simulink model "EMRAXDrive"  (R2023a)
settings: Solver=FixedStepAuto  StartTime=0.0  StopTime=emrax.stop_time  FixedStep=(1/6)*10^-05  RelTol=1e-3
PostLoadFcn:
  | motorFolder = fileparts(get_param('EMRAXDrive','FileName'));
  | run(fullfile(motorFolder,'MotorParameters.m'));
  | run(fullfile(motorFolder,'FlightParameters.m'));
  | emrax.flight_step = drone.step_s;
  | emrax.J = emrax.rotor_inertia + emrax.propeller_inertia;
  | emrax.current_limit = sqrt(2)*emrax.continuous_phase_arms; % amplitude-invariant dq, peak A
  | kt = 1.5*emrax.pole_pairs*emrax.flux;
  | current_bw = 2*pi*emrax.fsw/10;
  | inverter_gain = emrax.Vdc/2;
  | emrax.kp_d = current_bw*emrax.Ld/inverter_gain;
  | emrax.kp_q = current_bw*emrax.Lq/inverter_gain;
  | emrax.ki_i = current_bw*emrax.Rs/inverter_gain;
  | a = tand(65) + 1/cosd(65);
  | emrax.tau_filter = 1/(current_bw/100*a);
  | tau_total = emrax.tau_filter + 1/current_bw;
  | emrax.speed_kp = emrax.J/(kt*a*tau_total);
  | emrax.speed_ki = emrax.J/(kt*a^3*tau_total^2);
  | emrax.mission_start = emrax.ramp_seconds + emrax.settle_seconds;
  | 
  | emrax.stop_time = emrax.mission_start + drone.mission(end,1);
  | assignin('base','emrax',emrax);
  | scopePaths = find_system('EMRAXDrive/Drive results','BlockType','Scope'); for scopeIndex = 1:numel(scopePaths), scopeCfg = get_param(scopePaths{scopeIndex},'ScopeConfiguration'); scopeCfg.DataLoggingLimitDataPoints = false; scopeCfg.DataLoggingDecimateData = false; scopeCfg.TimeSpan = 'Auto'; scopeCfg.TimeDisplayOffset = '0'; scopeCfg.AxesScaling = 'Auto'; end;
InitFcn:
  | motorFolder = fileparts(get_param('EMRAXDrive','FileName'));
  | run(fullfile(motorFolder,'MotorParameters.m'));
  | run(fullfile(motorFolder,'FlightParameters.m'));
  | emrax.flight_step = drone.step_s;
  | emrax.J = emrax.rotor_inertia + emrax.propeller_inertia;
  | emrax.current_limit = sqrt(2)*emrax.continuous_phase_arms; % amplitude-invariant dq, peak A
  | kt = 1.5*emrax.pole_pairs*emrax.flux;
  | current_bw = 2*pi*emrax.fsw/10;
  | inverter_gain = emrax.Vdc/2;
  | emrax.kp_d = current_bw*emrax.Ld/inverter_gain;
  | emrax.kp_q = current_bw*emrax.Lq/inverter_gain;
  | emrax.ki_i = current_bw*emrax.Rs/inverter_gain;
  | a = tand(65) + 1/cosd(65);
  | emrax.tau_filter = 1/(current_bw/100*a);
  | tau_total = emrax.tau_filter + 1/current_bw;
  | emrax.speed_kp = emrax.J/(kt*a*tau_total);
  | emrax.speed_ki = emrax.J/(kt*a^3*tau_total^2);
  | emrax.mission_start = emrax.ramp_seconds + emrax.settle_seconds;
  | 
  | emrax.stop_time = emrax.mission_start + drone.mission(end,1);
  | assignin('base','emrax',emrax);
  | replayFile = fullfile(motorFolder,'Motor1Replay.mat');
  | assert(isfile(replayFile),'Open DroneFlight, press Run and wait for it to finish. Then press Run in EMRAXDrive.');
  | record = load(replayFile,'frontRightMotor');
  | assert(isfield(record,'frontRightMotor'),'Motor1Replay.mat has no motor signal. Run DroneFlight again.');
  | samples = record.frontRightMotor;
  | expected = (0:drone.step_s:drone.mission(end,1)).';
  | assert(isnumeric(samples) && isequal(size(samples),[3 numel(expected)]) && ...
  |     all(isfinite(samples),'all') && max(abs(samples(1,:).'-expected))<1e-8, ...
  |     'Motor1Replay.mat is incomplete or uses a different mission duration. Run DroneFlight to completion.');
  | t = samples(1,:).';
  | rpm = samples(2,:).';
  | loadNm = samples(3,:).';
  | assert(all(rpm>=0 & rpm<=emrax.speed_limit) && all(loadNm>=0),'Flight inputs exceed the selected drive limits.');
  | kT = drone.thrust_coefficient*drone.air_density_kg_m3*drone.diameter_m^4/(2*pi)^2;
  | hoverRPM = sqrt(drone.mass_kg*drone.gravity_m_s2/(drone.rotors*kT))*30/pi;
  | warm = (0:emrax.flight_step:emrax.mission_start-emrax.flight_step).';
  | fraction = min(warm/emrax.ramp_seconds,1);
  | time = [warm; t+emrax.mission_start];
  | emrax.stop_time = time(end);
  | speed = [hoverRPM*fraction; rpm];
  | torque = [loadNm(1)*fraction.^2; loadNm];
  | sourceTime = [time(1);time(1:end-1)+diff(time)/2];
  | assignin('base','shaft_speed_command',timeseries(speed,sourceTime));
  | assignin('base','shaft_load',timeseries(torque,sourceTime));
  | assignin('base','emrax',emrax);
libraries: spsIGBTDiodeLib x6, spsCurrentMeasurementLib x3, spsDCVoltageSourceLib x1, spsTriangleGeneratorLib x1, spsPermanentMagnetSynchronousMachineLib x1, sps_lib x1
settings Model: Creator=SUMANT  LastModifiedBy=SUMANT
settings DataIOCC: SaveOutput=off  SaveTime=off

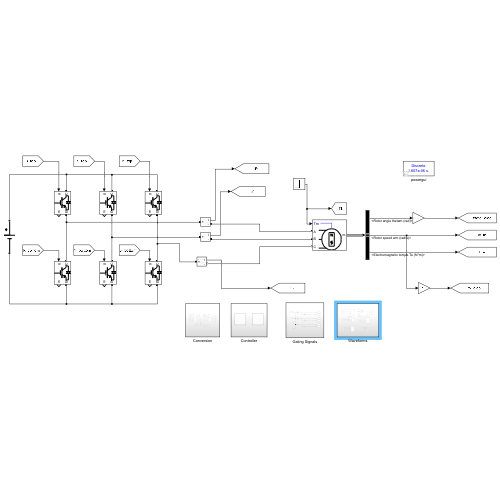
[thumbnail: Simulink's stored preview of the top-level diagram]
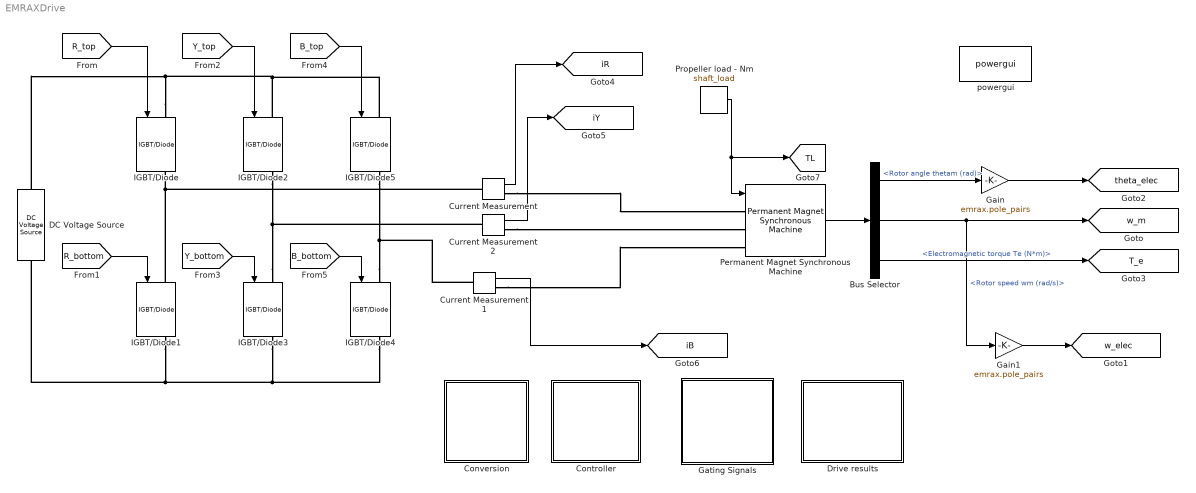
== system EMRAXDrive ==
  Bus Selector : BusSelector  OutputSignals=Rotor angle thetam (rad),Rotor speed wm (rad/s),Electromagnetic torque Te (N*m)
  Controller : Subsystem
  Conversion : Subsystem
  Current Measurement : spsCurrentMeasurementLib/Current Measurement  PhasorSimulation=off  OutputType=Complex  PSBequivalent=0
  Current Measurement1 : spsCurrentMeasurementLib/Current Measurement  PhasorSimulation=off  OutputType=Complex  PSBequivalent=0
  Current Measurement2 : spsCurrentMeasurementLib/Current Measurement  PhasorSimulation=off  OutputType=Complex  PSBequivalent=0
  DC Voltage Source : spsDCVoltageSourceLib/DC Voltage Source  Amplitude=emrax.Vdc  Measurements=None
  Gain : Gain  Gain=emrax.pole_pairs
  Gain1 : Gain  Gain=emrax.pole_pairs
  Gating Signals : Subsystem
  IGBT/Diode{,1..5} (6 alike) : spsIGBTDiodeLib/IGBT//Diode  Ron=1e-3  Rs=1e5  Cs=inf  Measurements=on
  Permanent Magnet Synchronous Machine : spsPermanentMagnetSynchronousMachineLib/Permanent Magnet Synchronous Machine  NbPhases=3  FluxDistribution=Sinusoidal  RotorType=Salient-pole  MechanicalLoad=Torque Tm  PresetModel=No  ShowDetailedParameters=on  MeasurementBus=off  Resistance=emrax.Rs  Inductance=8.5e-3  dqInductances=[emrax.Ld emrax.Lq]  La=0.000395  MachineConstant=Flux linkage established by magnets (V.s)  Flux=emrax.flux  VoltageCst=98.3079  TorqueCst=0.813  Flat=120  Mechanical=[emrax.J 0 emrax.pole_pairs 0]  PolePairs=emrax.pole_pairs  InitialConditions=[0,0, 0,0]  InitialConditions5ph=[0 0 0 0 0 0]  RefAngle=Aligned with phase A axis (original Park)  IterativeDiscreteModel=Trapezoidal non iterative  TsBlock=-1  TsPowergui=0
  Propeller load - Nm : FromWorkspace  VariableName=shaft_load  Interpolate=off  OutputAfterFinalValue=Holding final value  SampleTime=emrax.flight_step
  Drive results : Subsystem
  powergui : sps_lib/powergui  Priority=1  SimulationMode=Discrete  SampleTime=(1/6)*10^-05  frequency=60  Iterations=50  frequencyindice=0  Pbase=100e6  ErrMax=1e-4  UnitsV=kV  UnitsW=MW  buscounter=0  FunctionMessages=off  echomessages=off  EnableUseOfTLC=off  CurrentSourceSwitches=off  DisableSnubberDevices=off  DisableRonSwitches=off  DisableVfSwitches=off  DisplayEquations=off  AutomaticDiscreteSolvers=off  SolverType=Tustin/Backward Euler (TBE)  Interpol=off  ExternalGateDelay=off  methode=off  Ts=100  x0status=blocks  SPID=on  SwTol=0  HookPort=off  NonlinearTolerance=1e-4  nMaxIteration=100  ContinueOnMaxIteration=off  RestoreLinks=warning  ResistiveCurrentMeasurement=off  Frange=[0:2:500]  Ylog=off  Xlog=on  ShowGrid=off  save=off  variable=ZData  structure=0  ZoomFFT=off  StartTime=0.0  cycles=1  DisplayStyle=1  fundamental=60  FreqAxis=off  MaxFrequency=1000  frequencyindicesteady=1  RmsSteady=1  display=off
  tag scope: TL=global, T_e=global, iB=global, iR=global, iY=global, theta_elec=global, w_elec=global, w_m=global
  wires:
  Propeller load - Nm/1 -> [TL], Permanent Magnet Synchronous Machine/1
  [B_bottom] -> IGBT/Diode4/1
  Current Measurement/1 -> [iR]
  Bus Selector/3 -> [T_e]  "<Electromagnetic torque Te (N*m)>"
  [R_bottom] -> IGBT/Diode1/1
  Gain1/1 -> [w_elec]
  Bus Selector/2 -> Gain1/1, [w_m]  "<Rotor speed wm (rad/s)>"
  Gain/1 -> [theta_elec]
  [Y_bottom] -> IGBT/Diode3/1
  Bus Selector/1 -> Gain/1  "<Rotor angle thetam (rad)>"
  Current Measurement1/1 -> [iB]
  [Y_top] -> IGBT/Diode2/1
  Current Measurement2/1 -> [iY]
  [R_top] -> IGBT/Diode/1
  Permanent Magnet Synchronous Machine/1 -> Bus Selector/1
  [B_top] -> IGBT/Diode5/1
  connections:
  IGBT/Diode4/LConn1 -- IGBT/Diode5/RConn1 -- Current Measurement1/LConn1
  Current Measurement/LConn1 -- IGBT/Diode1/LConn1 -- IGBT/Diode/RConn1
  DC Voltage Source/LConn1 -- IGBT/Diode1/RConn1 -- IGBT/Diode3/RConn1 -- IGBT/Diode4/RConn1
  IGBT/Diode3/LConn1 -- IGBT/Diode2/RConn1 -- Current Measurement2/LConn1
  IGBT/Diode/LConn1 -- DC Voltage Source/RConn1 -- IGBT/Diode5/LConn1 -- IGBT/Diode2/LConn1
  Current Measurement/RConn1 -- Permanent Magnet Synchronous Machine/LConn1
  Current Measurement2/RConn1 -- Permanent Magnet Synchronous Machine/LConn2
  Current Measurement1/RConn1 -- Permanent Magnet Synchronous Machine/LConn3

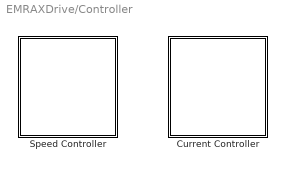
== system EMRAXDrive/Controller ==
  Current Controller : Subsystem
  Speed Controller : Subsystem

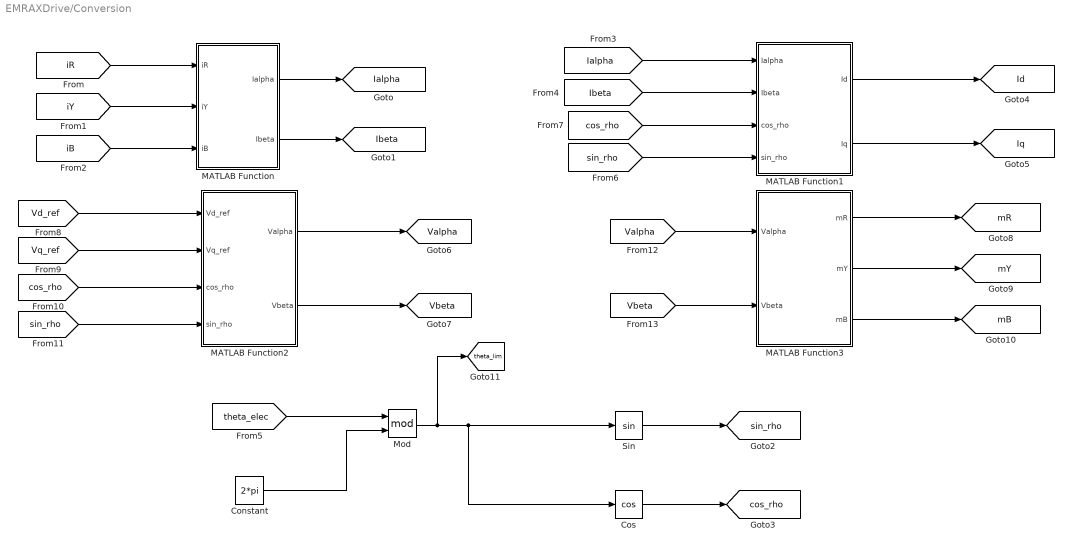
== system EMRAXDrive/Conversion ==
  Constant : Constant  Value=2*pi
  Cos : Trigonometry  Operator=cos
  MATLAB Function : MATLAB Function  TreatAsAtomicUnit=on
  MATLAB Function1 : MATLAB Function  TreatAsAtomicUnit=on
  MATLAB Function2 : MATLAB Function  TreatAsAtomicUnit=on
  MATLAB Function3 : MATLAB Function  TreatAsAtomicUnit=on
  Mod : Math  Operator=mod
  Sin : Trigonometry
  tag scope: Ialpha=global, Ibeta=global, Id=global, Iq=global, Valpha=global, Vbeta=global, cos_rho=global, mB=global, mR=global, mY=global, sin_rho=global, theta_lim=global
  wires:
  [iR] -> MATLAB Function/1(iR)
  [iB] -> MATLAB Function/3(iB)
  [iY] -> MATLAB Function/2(iY)
  MATLAB Function/1(Ialpha) -> [Ialpha]
  MATLAB Function/2(Ibeta) -> [Ibeta]
  [Ialpha] -> MATLAB Function1/1(Ialpha)
  [Ibeta] -> MATLAB Function1/2(Ibeta)
  [theta_elec] -> Mod/1
  Constant/1 -> Mod/2
  Mod/1 -> [theta_lim], Cos/1, Sin/1
  Sin/1 -> [sin_rho]
  [sin_rho] -> MATLAB Function1/4(sin_rho)
  Cos/1 -> [cos_rho]
  [cos_rho] -> MATLAB Function1/3(cos_rho)
  MATLAB Function1/1(Id) -> [Id]
  MATLAB Function1/2(Iq) -> [Iq]
  [Vd_ref] -> MATLAB Function2/1(Vd_ref)
  [Vq_ref] -> MATLAB Function2/2(Vq_ref)
  [cos_rho] -> MATLAB Function2/3(cos_rho)
  [sin_rho] -> MATLAB Function2/4(sin_rho)
  MATLAB Function2/2(Vbeta) -> [Vbeta]
  MATLAB Function2/1(Valpha) -> [Valpha]
  [Valpha] -> MATLAB Function3/1(Valpha)
  [Vbeta] -> MATLAB Function3/2(Vbeta)
  MATLAB Function3/1(mR) -> [mR]
  MATLAB Function3/2(mY) -> [mY]
  MATLAB Function3/3(mB) -> [mB]

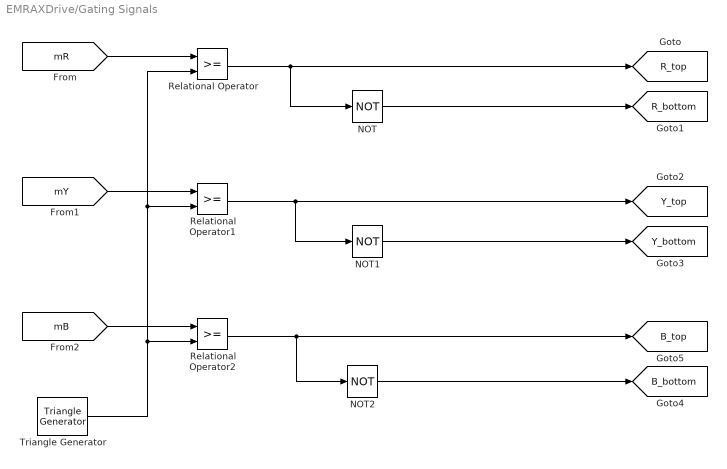
== system EMRAXDrive/Gating Signals ==
  NOT : Logic  Operator=NOT  IconShape=distinctive  AllPortsSameDT=off  OutDataTypeStr=boolean
  NOT1 : Logic  Operator=NOT  IconShape=distinctive  AllPortsSameDT=off  OutDataTypeStr=boolean
  NOT2 : Logic  Operator=NOT  IconShape=distinctive  AllPortsSameDT=off  OutDataTypeStr=boolean
  Relational Operator : RelationalOperator  OutDataTypeStr=boolean  RndMeth=Simplest  InputSameDT=off
  Relational Operator1 : RelationalOperator  OutDataTypeStr=boolean  RndMeth=Simplest  InputSameDT=off
  Relational Operator2 : RelationalOperator  OutDataTypeStr=boolean  RndMeth=Simplest  InputSameDT=off
  Triangle Generator : spsTriangleGeneratorLib/Triangle Generator  Freq=emrax.fsw  Phase=90  Ts=0
  tag scope: B_bottom=global, B_top=global, R_bottom=global, R_top=global, Y_bottom=global, Y_top=global
  wires:
  [mB] -> Relational Operator2/1
  [mY] -> Relational Operator1/1
  [mR] -> Relational Operator/1
  Triangle Generator/1 -> Relational Operator2/2, Relational Operator1/2, Relational Operator/2
  Relational Operator/1 -> NOT/1, [R_top]
  Relational Operator2/1 -> NOT2/1, [B_top]
  NOT2/1 -> [B_bottom]
  NOT1/1 -> [Y_bottom]
  Relational Operator1/1 -> NOT1/1, [Y_top]
  NOT/1 -> [R_bottom]

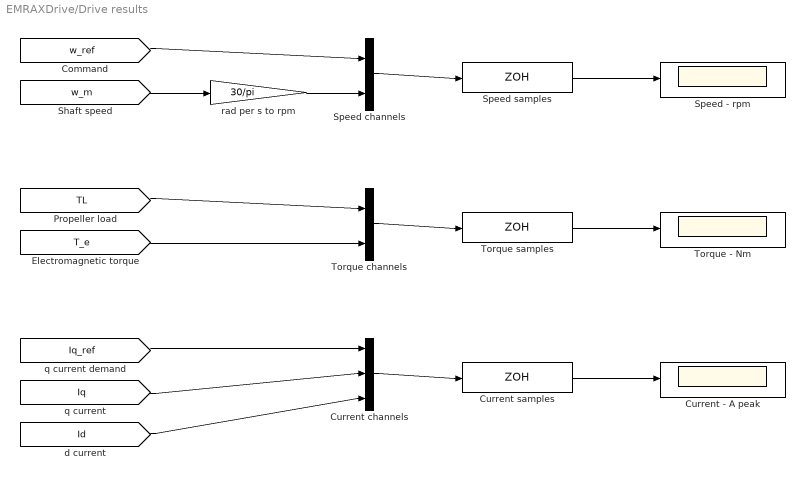
== system EMRAXDrive/Drive results ==
  rad per s to rpm : Gain  Gain=30/pi
  Speed channels : Mux  Inputs=2
  Speed samples : ZeroOrderHold  SampleTime=emrax.flight_step
  Speed - rpm : Scope
      settings: OpenAtSimulationStart=off
  Torque channels : Mux  Inputs=2
  Torque samples : ZeroOrderHold  SampleTime=emrax.flight_step
  Torque - Nm : Scope
      settings: OpenAtSimulationStart=off
  Current channels : Mux  Inputs=3
  Current samples : ZeroOrderHold  SampleTime=emrax.flight_step
  Current - A peak : Scope
      settings: OpenAtSimulationStart=off
  wires:
  [w_m] -> rad per s to rpm/1
  [w_ref] -> Speed channels/1
  rad per s to rpm/1 -> Speed channels/2
  Speed channels/1 -> Speed samples/1
  Speed samples/1 -> Speed - rpm/1
  [TL] -> Torque channels/1
  [T_e] -> Torque channels/2
  Torque channels/1 -> Torque samples/1
  Torque samples/1 -> Torque - Nm/1
  [Iq_ref] -> Current channels/1
  [Iq] -> Current channels/2
  [Id] -> Current channels/3
  Current channels/1 -> Current samples/1
  Current samples/1 -> Current - A peak/1

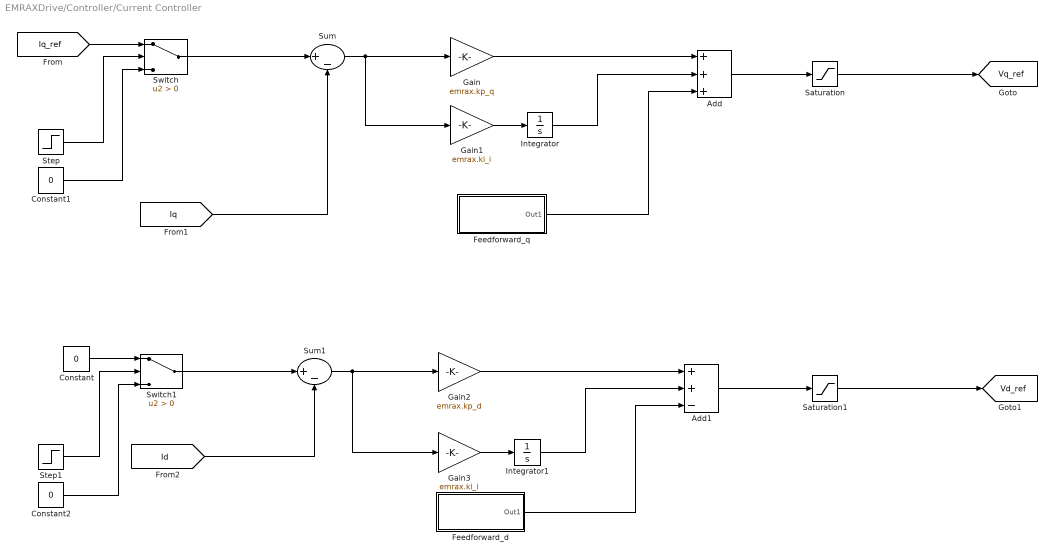
== system EMRAXDrive/Controller/Current Controller ==
  Add : Sum  Inputs=+++
  Add1 : Sum  Inputs=++-
  Constant : Constant  Value=0
  Constant1 : Constant  Value=0
  Constant2 : Constant  Value=0
  Feedforward_d : Subsystem
  Feedforward_q : Subsystem
  Gain : Gain  Gain=emrax.kp_q
  Gain1 : Gain  Gain=emrax.ki_i
  Gain2 : Gain  Gain=emrax.kp_d
  Gain3 : Gain  Gain=emrax.ki_i
  Integrator : Integrator  LimitOutput=on  UpperSaturationLimit=1  LowerSaturationLimit=-1
  Integrator1 : Integrator  LimitOutput=on  UpperSaturationLimit=1  LowerSaturationLimit=-1
  Saturation : Saturate  UpperLimit=1  LowerLimit=-1
  Saturation1 : Saturate  UpperLimit=1  LowerLimit=-1
  Step : Step  Time=0  SampleTime=0
  Step1 : Step  Time=0  SampleTime=0
  Sum : Sum  Inputs=|+-
  Sum1 : Sum  Inputs=|+-
  Switch : Switch  Criteria=u2 > Threshold  SaturateOnIntegerOverflow=off  InputSameDT=off
  Switch1 : Switch  Criteria=u2 > Threshold  SaturateOnIntegerOverflow=off  InputSameDT=off
  tag scope: Vd_ref=global, Vq_ref=global
  wires:
  [Iq] -> Sum/2
  Sum/1 -> Gain/1, Gain1/1
  Gain1/1 -> Integrator/1
  Gain/1 -> Add/1
  Feedforward_q/1(Out1) -> Add/3
  Integrator/1 -> Add/2
  Add/1 -> Saturation/1
  Saturation/1 -> [Vq_ref]
  Switch1/1 -> Sum1/1
  [Id] -> Sum1/2
  Gain2/1 -> Add1/1
  Feedforward_d/1(Out1) -> Add1/3
  Sum1/1 -> Gain3/1, Gain2/1
  Integrator1/1 -> Add1/2
  Gain3/1 -> Integrator1/1
  Saturation1/1 -> [Vd_ref]
  Add1/1 -> Saturation1/1
  [Iq_ref] -> Switch/1
  Switch/1 -> Sum/1
  Step/1 -> Switch/2
  Constant1/1 -> Switch/3
  Constant/1 -> Switch1/1
  Constant2/1 -> Switch1/3
  Step1/1 -> Switch1/2

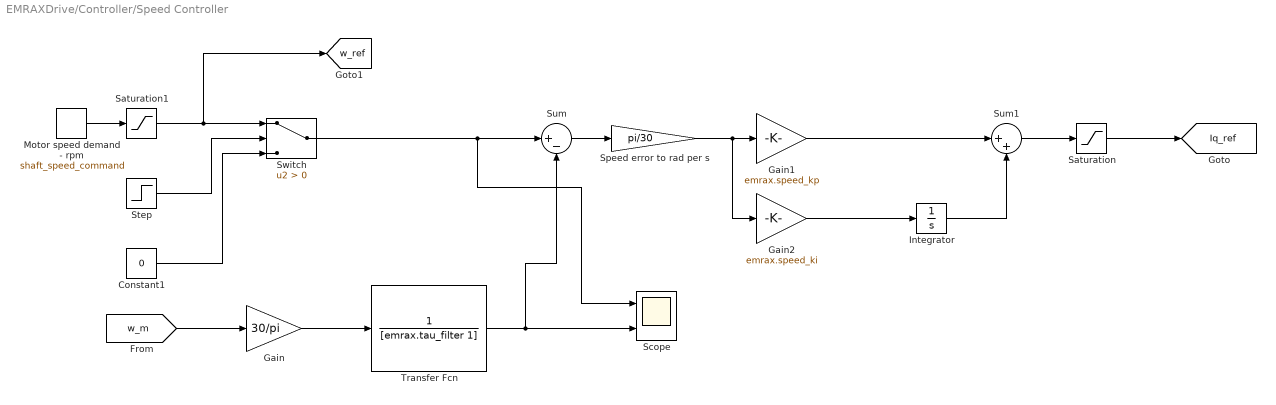
== system EMRAXDrive/Controller/Speed Controller ==
  Constant1 : Constant  Value=0
  Gain : Gain  Gain=30/pi
  Gain1 : Gain  Gain=emrax.speed_kp
  Gain2 : Gain  Gain=emrax.speed_ki
  Integrator : Integrator  LimitOutput=on  UpperSaturationLimit=emrax.current_limit  LowerSaturationLimit=-emrax.current_limit
  Motor speed demand - rpm : FromWorkspace  VariableName=shaft_speed_command  Interpolate=off  OutputAfterFinalValue=Holding final value  SampleTime=emrax.flight_step
  Saturation : Saturate  UpperLimit=emrax.current_limit  LowerLimit=-emrax.current_limit
  Saturation1 : Saturate  UpperLimit=emrax.speed_limit  LowerLimit=-emrax.speed_limit
  Scope : Scope  NumInputPorts=2
  Step : Step  SampleTime=0  Time=0
  Sum : Sum  Inputs=|+-
  Sum1 : Sum  Inputs=|++
  Switch : Switch  Criteria=u2 > Threshold  SaturateOnIntegerOverflow=off  InputSameDT=off
  Transfer Fcn : TransferFcn  Denominator=[emrax.tau_filter 1]
  Speed error to rad per s : Gain  Gain=pi/30
  tag scope: Iq_ref=global, w_ref=global
  wires:
  [w_m] -> Gain/1
  Gain/1 -> Transfer Fcn/1
  Switch/1 -> Scope/1, Sum/1
  Transfer Fcn/1 -> Sum/2, Scope/2
  Speed error to rad per s/1 -> Gain2/1, Gain1/1
  Gain2/1 -> Integrator/1
  Gain1/1 -> Sum1/1
  Integrator/1 -> Sum1/2
  Sum1/1 -> Saturation/1
  Saturation/1 -> [Iq_ref]
  Step/1 -> Switch/2
  Constant1/1 -> Switch/3
  Saturation1/1 -> [w_ref], Switch/1
  Motor speed demand - rpm/1 -> Saturation1/1
  Sum/1 -> Speed error to rad per s/1

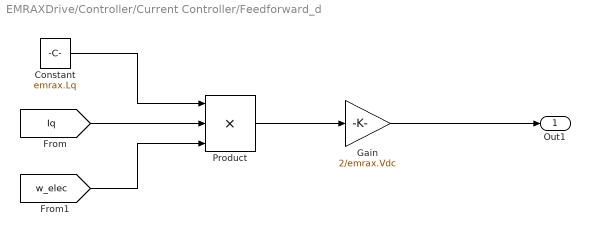
== system EMRAXDrive/Controller/Current Controller/Feedforward_d ==
  Constant : Constant  Value=emrax.Lq
  Gain : Gain  Gain=2/emrax.Vdc
  Product : Product  Inputs=3
  Out1 : Outport
  wires:
  Constant/1 -> Product/1
  [w_elec] -> Product/3
  [Iq] -> Product/2
  Product/1 -> Gain/1
  Gain/1 -> Out1/1

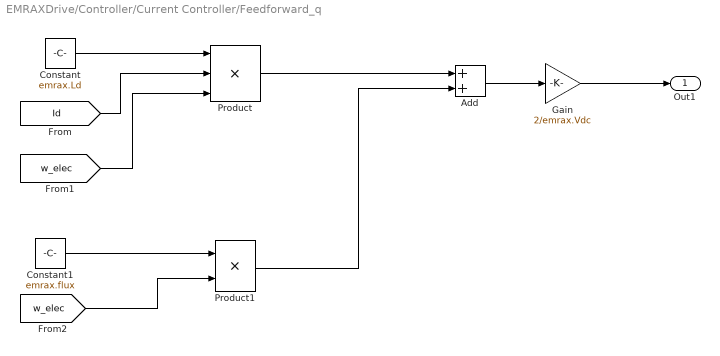
== system EMRAXDrive/Controller/Current Controller/Feedforward_q ==
  Add : Sum
  Constant : Constant  Value=emrax.Ld
  Constant1 : Constant  Value=emrax.flux
  Gain : Gain  Gain=2/emrax.Vdc
  Product : Product  Inputs=3
  Product1 : Product
  Out1 : Outport
  wires:
  Constant/1 -> Product/1
  [Id] -> Product/2
  [w_elec] -> Product/3
  Constant1/1 -> Product1/1
  [w_elec] -> Product1/2
  Product/1 -> Add/1
  Product1/1 -> Add/2
  Add/1 -> Gain/1
  Gain/1 -> Out1/1

== matlab function EMRAXDrive/Conversion/MATLAB Function1 ==
  data: Ialpha input; Id output; Ibeta input; cos_rho input; Iq output; sin_rho input
function [Id,Iq] = fcn(Ialpha,Ibeta,cos_rho,sin_rho)

Id= Ialpha*(cos_rho)+Ibeta*(sin_rho);
Iq=-Ialpha*(sin_rho)+Ibeta*(cos_rho);

== matlab function EMRAXDrive/Conversion/MATLAB Function ==
  data: iR input; Ialpha output; iY input; iB input; Ibeta output
function [Ialpha,Ibeta] = fcn(iR,iY,iB)
Ialpha = (2/3)*(iR - (iY+iB)/2);
Ibeta = (iY-iB)/sqrt(3);

== matlab function EMRAXDrive/Conversion/MATLAB Function2 ==
  data: Vd_ref input; Valpha output; Vq_ref input; cos_rho input; Vbeta output; sin_rho input
function [Valpha,Vbeta] = fcn(Vd_ref,Vq_ref,cos_rho,sin_rho)

Valpha=Vd_ref*(cos_rho)-Vq_ref*(sin_rho);
Vbeta=Vd_ref*(sin_rho)+Vq_ref*(cos_rho);

== matlab function EMRAXDrive/Conversion/MATLAB Function3 ==
  data: Valpha input; mR output; Vbeta input; mY output; mB output
function [mR,mY,mB] = fcn(Valpha,Vbeta)
% Linear sinusoidal PWM. Limit the rotating voltage vector to Vdc/2.
scale = max(1,hypot(Valpha,Vbeta));
a = Valpha/scale;
b = Vbeta/scale;
mR = a;
mY = -a/2 + sqrt(3)*b/2;
mB = -a/2 - sqrt(3)*b/2;
